simulink model "SMTorqueControl_AI"  (R2026a)
settings: Solver=FixedStepDiscrete  StopTime=1  FixedStep=Ts  EnableMultiTasking=on
PreLoadFcn:
  | if exist(fullfile(pwd, 'Ortak_Veri_ve_Parametreler'), 'dir'), addpath(fullfile(pwd, 'Ortak_Veri_ve_Parametreler')); end
  | if exist(fullfile(pwd, '..', 'Ortak_Veri_ve_Parametreler'), 'dir'), addpath(fullfile(pwd, '..', 'Ortak_Veri_ve_Parametreler')); end
  | if exist(fullfile(pwd, 'Mat_Dosyalari'), 'dir'), addpath(fullfile(pwd, 'Mat_Dosyalari')); end
  | SMTorqueControlData;
InitFcn:
  | if exist(fullfile(pwd, 'Ortak_Veri_ve_Parametreler'), 'dir'), addpath(fullfile(pwd, 'Ortak_Veri_ve_Parametreler')); end
  | if exist(fullfile(pwd, '..', 'Ortak_Veri_ve_Parametreler'), 'dir'), addpath(fullfile(pwd, '..', 'Ortak_Veri_ve_Parametreler')); end
  | if exist(fullfile(pwd, 'Mat_Dosyalari'), 'dir'), addpath(fullfile(pwd, 'Mat_Dosyalari')); end
  | SMTorqueControlData;
undefined symbols (not defined in the file): denZC_id, denZC_if, denZC_iq, ee_sli_rtmsupport, fsw, gcbh, Ibase, ID_MAP, IF_MAP, Ifbase, IQ_MAP, Kaw_id, Kaw_if, Kaw_iq, Ki_id, Ki_if, Ki_iq, Kp_id, Kp_if, Kp_iq, L_base, Lad, Ld, Lq, numZC_id, numZC_if, numZC_iq, p, Pmax, RPM_VECT, Tbase, TQ_VECT, Ts, Tsi, VDC_VECT, Vnom
libraries: nesl_utility x16, fl_lib x11, ee_lib x6, eeGeneralControl x3, eeTransforms x2, deeplib x2, sl_discontinuities x2, SignalEditorBlockLib x2, eeDqVoltageLimiter x1, simulink x1, sl_signal_attributes x1, eePwmGenerator x1
(part 2 of 2)

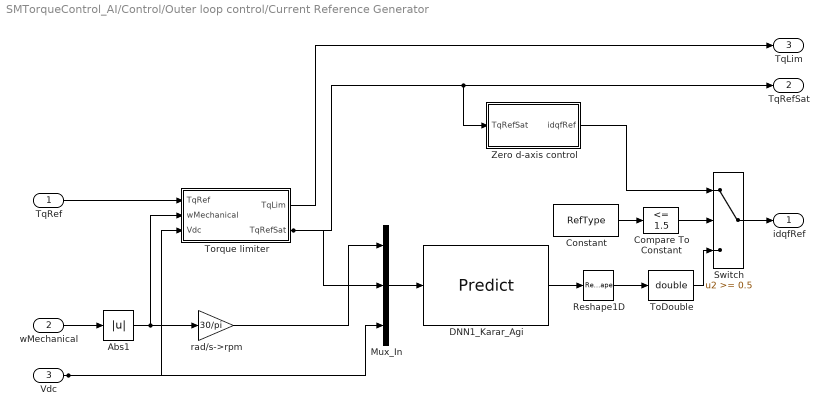
== system SMTorqueControl_AI/Control/Outer loop control/Current Reference Generator ==
  TqRef : Inport  SampleTime=Ts
  wMechanical : Inport  Port=2  SampleTime=Ts
  Vdc : Inport  Port=3  SampleTime=Ts
  Abs1 : Abs  SaturateOnIntegerOverflow=off
  Compare To Constant : simulink/Logic and Bit Operations/Compare To Constant  relop=<=  const=1.5  OutDataTypeStr=boolean
  Constant : Constant  Value=RefType  SampleTime=Ts
  DNN1_Karar_Agi : deeplib/Predict  Network=Network from MAT-file  NetworkFunction=squeezenet  NetworkFilePath=DNN1_DecisionNet.mat  MiniBatchSize=128  SimulateUsing=Interpreted execution  InputDataFormats={'Giris', 'CB';}  Predictions=on  Activations={}  ForceInterpretedSim=off  EnableDLNetwork=on  LastKnownNetworkFilePath='C:\Users\Dogukan.kilinc\OneDrive - figes.com.tr\Documents\MATLAB\Examples\R2026a\simscapeelectrical\SMTorqueControlExample\Mat_Dosyalari\DNN1_DecisionNet.mat'  LastKnownNetworkTimeStamp=740288.500960648176260292530059814453125
  Mux_In : Mux  Inputs=3
  Reshape1D : Reshape
  Switch : Switch  Threshold=0.5  SaturateOnIntegerOverflow=off  InputSameDT=off
  ToDouble : DataTypeConversion  OutDataTypeStr=double  SaturateOnIntegerOverflow=off  RndMeth=Floor
  Torque limiter : Subsystem
  Zero d-axis control : Subsystem
  rad/s->rpm : Gain  Gain=30/pi
  idqfRef : Outport  VectorParamsAs1DForOutWhenUnconnected=off
  TqRefSat : Outport  Port=2  VectorParamsAs1DForOutWhenUnconnected=off
  TqLim : Outport  Port=3  VectorParamsAs1DForOutWhenUnconnected=off
  wires:
  Compare To Constant/1 -> Switch/2
  Zero d-axis control/1(idqfRef) -> Switch/1
  Torque limiter/2(TqRefSat) -> TqRefSat/1, Zero d-axis control/1(TqRefSat), Mux_In/2
  Torque limiter/1(TqLim) -> TqLim/1
  Abs1/1 -> Torque limiter/2(wMechanical), rad/s->rpm/1
  Switch/1 -> idqfRef/1
  TqRef/1 -> Torque limiter/1(TqRef)
  wMechanical/1 -> Abs1/1
  Vdc/1 -> Torque limiter/3(Vdc), Mux_In/3
  Constant/1 -> Compare To Constant/1
  rad/s->rpm/1 -> Mux_In/1
  Mux_In/1 -> DNN1_Karar_Agi/1
  DNN1_Karar_Agi/1 -> Reshape1D/1
  Reshape1D/1 -> ToDouble/1
  ToDouble/1 -> Switch/3

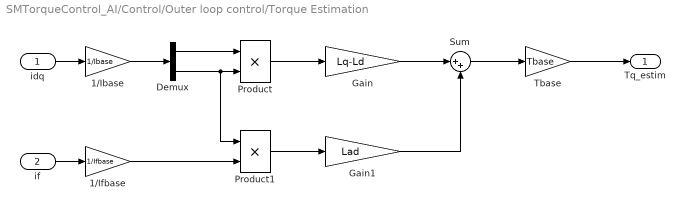
== system SMTorqueControl_AI/Control/Outer loop control/Torque Estimation ==
  idq : Inport
  if : Inport  Port=2
  1/Ibase : Gain  Gain=1/Ibase
  1/Ifbase : Gain  Gain=1/Ifbase
  Demux : Demux  Outputs=2
  Gain : Gain  Gain=Lq-Ld
  Gain1 : Gain  Gain=Lad
  Product : Product
  Product1 : Product
  Sum : Sum  Inputs=|++
  Tbase : Gain  Gain=Tbase
  Tq_estim : Outport  VectorParamsAs1DForOutWhenUnconnected=off
  wires:
  idq/1 -> 1/Ibase/1
  Demux/1 -> Product/1
  Product/1 -> Gain/1
  Gain/1 -> Sum/1
  Demux/2 -> Product1/1, Product/2
  Product1/1 -> Gain1/1
  Sum/1 -> Tbase/1
  if/1 -> 1/Ifbase/1
  1/Ifbase/1 -> Product1/2
  1/Ibase/1 -> Demux/1
  Tbase/1 -> Tq_estim/1
  Gain1/1 -> Sum/2

== system SMTorqueControl_AI/Control/Current control/SM Current Controller/vf limiter ==
  vfUnsat : Inport
  VfMax : Inport  Port=2
  Saturation Dynamic1 : sl_discontinuities/Saturation Dynamic  OutMin=[]  OutMax=[]  OutDataTypeStr=Inherit: Same as second input  OutDataType=fixdt(1, 16)  OutScaling=2^-10  DoSatur=off
  "Sign Change " : Gain  Gain=-1
  vfRef : Outport  VectorParamsAs1DForOutWhenUnconnected=off
  wires:
  Saturation Dynamic1/1 -> vfRef/1
  "Sign Change "/1 -> Saturation Dynamic1/3
  VfMax/1 -> "Sign Change "/1, Saturation Dynamic1/1
  vfUnsat/1 -> Saturation Dynamic1/2

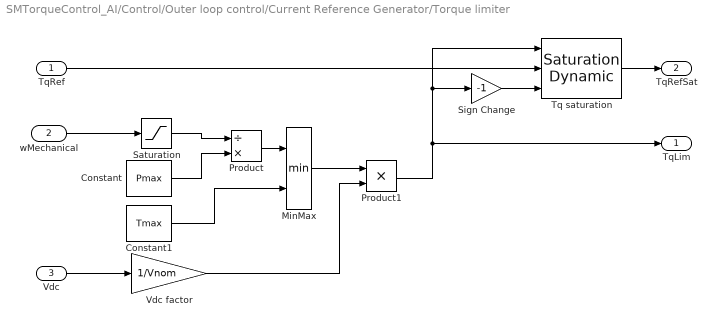
== system SMTorqueControl_AI/Control/Outer loop control/Current Reference Generator/Torque limiter ==
  TqRef : Inport
  wMechanical : Inport  Port=2
  Vdc : Inport  Port=3
  Constant : Constant  Value=Pmax  SampleTime=Ts
  Constant1 : Constant  Value=Tmax  SampleTime=Ts
  MinMax : MinMax  Inputs=2  OutDataTypeStr=Inherit: Same as first input
  Product : Product  Inputs=/*  OutDataTypeStr=Inherit: Same as first input
  Product1 : Product
  Saturation : Saturate  UpperLimit=inf  LowerLimit=Pmax/Tmax
  Sign Change : Gain  Gain=-1
  Tq saturation : sl_discontinuities/Saturation Dynamic  OutMin=[]  OutMax=[]  OutDataTypeStr=Inherit: Same as second input  OutDataType=fixdt(1, 16)  OutScaling=2^-10  DoSatur=off
  Vdc factor : Gain  Gain=1/Vnom
  TqLim : Outport  VectorParamsAs1DForOutWhenUnconnected=off
  TqRefSat : Outport  Port=2  VectorParamsAs1DForOutWhenUnconnected=off
  wires:
  Constant/1 -> Product/2
  Saturation/1 -> Product/1
  Tq saturation/1 -> TqRefSat/1
  Product1/1 -> Tq saturation/1, Sign Change/1, TqLim/1
  TqRef/1 -> Tq saturation/2
  Vdc/1 -> Vdc factor/1
  Constant1/1 -> MinMax/2
  wMechanical/1 -> Saturation/1
  Product/1 -> MinMax/1
  Sign Change/1 -> Tq saturation/3
  MinMax/1 -> Product1/1
  Vdc factor/1 -> Product1/2

== system SMTorqueControl_AI/Control/Outer loop control/Current Reference Generator/Zero d-axis control ==
  TqRefSat : Inport
  Abs : Abs  SaturateOnIntegerOverflow=off
  Data Type Conversion Inherited : sl_signal_attributes/Data Type Conversion Inherited  ConvertRealWorld=Real World Value  DoSatur=off
  Ifmin : Constant  Value=0.01*ifmax  SampleTime=Ts
  Kt : Gain  Gain=Kt
  MinMax : MinMax  Function=max  Inputs=2  OutDataTypeStr=Inherit: Same as first input
  Mux1 : Mux  Inputs=3
  Product : Product  Inputs=*/
  idRef : Constant  Value=0  SampleTime=Ts
  ifmax/Tmax : Gain  Gain=ifmax/Tmax
  idqfRef : Outport  VectorParamsAs1DForOutWhenUnconnected=off
  wires:
  idRef/1 -> Data Type Conversion Inherited/2
  Data Type Conversion Inherited/1 -> Mux1/1
  Ifmin/1 -> MinMax/2
  MinMax/1 -> Mux1/3, Kt/1
  Kt/1 -> Product/2
  ifmax/Tmax/1 -> MinMax/1
  Abs/1 -> ifmax/Tmax/1
  TqRefSat/1 -> Abs/1, Data Type Conversion Inherited/1, Product/1
  Product/1 -> Mux1/2
  Mux1/1 -> idqfRef/1

== stateflow chart SMTorqueControl_AI/Control/Task scheduler ==
  (default) -> (junction 23) : CLK_50us
  (junction 23) -> (junction 17)
  (junction 17) -> (junction 22) [order 2]
  (junction 17) -> (junction 22) [order 1] : [cnt%%2==0]{Task_100us_1;}
  (junction 22) -> (junction 18) [order 2]
  (junction 22) -> (junction 18) [order 1] : [cnt%%2==0]{Task_100us_2;}
  (junction 18) -> (junction 21) [order 1] : [cnt%%20==0]{Task_1ms_1;}
  (junction 18) -> (junction 21) [order 2]
  (junction 21) -> (junction 34) [order 2]
  (junction 21) -> (junction 16) [order 1] : [1]{cnt++;}
  data: cnt local int32
  events: Task_100us_1 output FUNCTION_CALL_EVENT; Task_100us_2 output FUNCTION_CALL_EVENT; Task_1ms_1 output FUNCTION_CALL_EVENT; CLK_50us input FUNCTION_CALL_EVENT
